simulink model "Buck_28V_12V_Analysis"  (R2023a)
settings: Solver=ode23t  StartTime=0.0  StopTime=0.05  MaxStep=1e-6  RelTol=1e-3
undefined symbols (not defined in the file): Rload
libraries: ee_lib x34, nesl_utility x33, fl_lib x26, simulink x24, slpidlib x4, simulink_extras x3
(part 2 of 2)

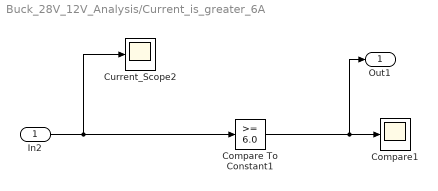
== system Buck_28V_12V_Analysis/Current_is_greater_6A ==
  In2 : Inport
  Compare To Constant1 : simulink/Logic and Bit Operations/Compare To Constant  relop=>=  const=6.0  OutDataTypeStr=boolean  ZeroCross=off
  Compare1 : Scope
  Current_Scope2 : Scope
  Out1 : Outport
  wires:
  Compare To Constant1/1 -> Out1/1, Compare1/1
  In2/1 -> Compare To Constant1/1, Current_Scope2/1

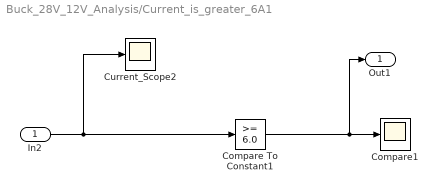
== system Buck_28V_12V_Analysis/Current_is_greater_6A1 ==
  In2 : Inport
  Compare To Constant1 : simulink/Logic and Bit Operations/Compare To Constant  relop=>=  const=6.0  OutDataTypeStr=boolean  ZeroCross=off
  Compare1 : Scope
  Current_Scope2 : Scope
  Out1 : Outport
  wires:
  In2/1 -> Current_Scope2/1, Compare To Constant1/1
  Compare To Constant1/1 -> Compare1/1, Out1/1

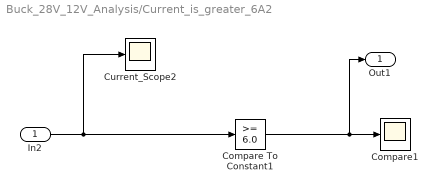
== system Buck_28V_12V_Analysis/Current_is_greater_6A2 ==
  In2 : Inport
  Compare To Constant1 : simulink/Logic and Bit Operations/Compare To Constant  relop=>=  const=6.0  OutDataTypeStr=boolean  ZeroCross=off
  Compare1 : Scope
  Current_Scope2 : Scope
  Out1 : Outport
  wires:
  In2/1 -> Current_Scope2/1, Compare To Constant1/1
  Compare To Constant1/1 -> Compare1/1, Out1/1

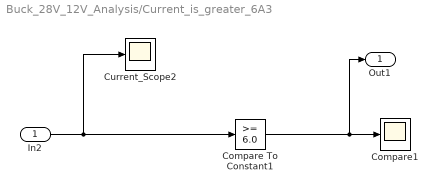
== system Buck_28V_12V_Analysis/Current_is_greater_6A3 ==
  In2 : Inport
  Compare To Constant1 : simulink/Logic and Bit Operations/Compare To Constant  relop=>=  const=6.0  OutDataTypeStr=boolean  ZeroCross=off
  Compare1 : Scope
  Current_Scope2 : Scope
  Out1 : Outport
  wires:
  In2/1 -> Current_Scope2/1, Compare To Constant1/1
  Compare To Constant1/1 -> Compare1/1, Out1/1

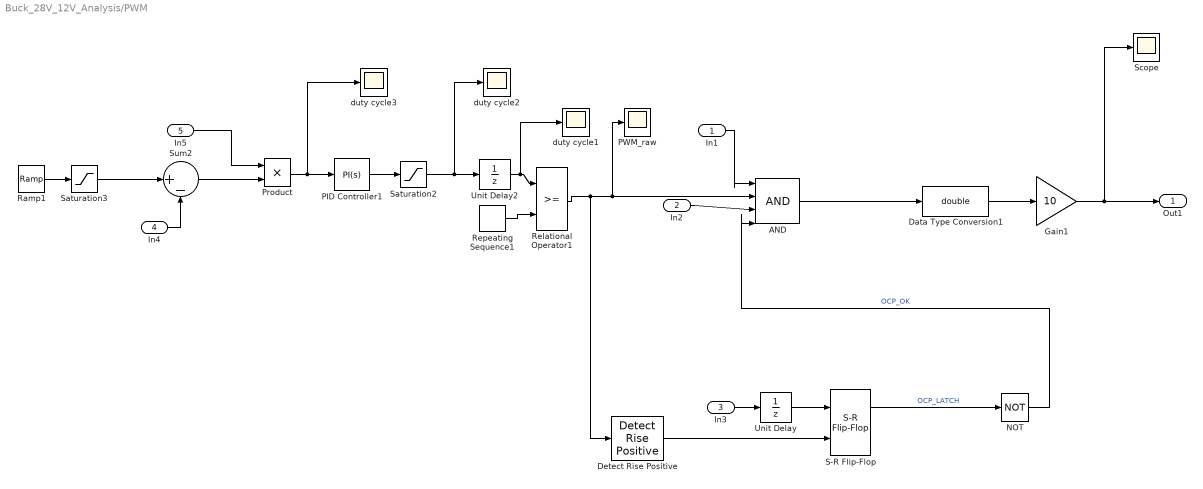
== system Buck_28V_12V_Analysis/PWM ==
  In1 : Inport
  In2 : Inport  Port=2
  In3 : Inport  Port=3
  In4 : Inport  Port=4
  In5 : Inport  Port=5
  AND : Logic  Inputs=4  IconShape=distinctive  AllPortsSameDT=off  OutDataTypeStr=boolean
  Data Type Conversion1 : DataTypeConversion  OutDataTypeStr=double  SaturateOnIntegerOverflow=off  RndMeth=Floor
  Detect Rise Positive : simulink/Logic and Bit Operations/Detect Rise Positive  vinit=0  OutDataTypeStr=boolean
  Gain1 : Gain  Gain=10
  NOT : Logic  Operator=NOT  IconShape=distinctive  AllPortsSameDT=off  OutDataTypeStr=boolean
  PID Controller1 : slpidlib/PID Controller  Controller=PI  Form=Parallel  TimeDomain=Continuous-time  UseExternalTs=off  SampleTime=-1  IntegratorMethod=Forward Euler  FilterMethod=Forward Euler  ControllerParametersSource=internal  P=0.02  I=50  UseKiTs=off  D=0  N=100  UseFilter=on  TunerSelectOption=Transfer Function Based (PID Tuner App)  ZeroCross=off  InitialConditionSource=internal  InitialConditionForIntegrator=0  InitialConditionForFilter=0  DifferentiatorICPrevScaledInput=0  ExternalReset=none  TrackingMode=off  Kt=1  LimitOutput=off  SatLimitsSource=internal  UpperSaturationLimit=inf  LowerSaturationLimit=-inf  LinearizeAsGain=on  AntiWindupMode=none  Kb=1  LimitIntegrator=off  UpperIntegratorSaturationLimit=inf  LowerIntegratorSaturationLimit=-inf  POutMin=[]  POutMax=[]  IOutMin=[]  IOutMax=[]  DOutMin=[]  DOutMax=[]  NOutMin=[]  NOutMax=[]  SumOutMin=[]  SumOutMax=[]  SaturationOutMin=[]  SaturationOutMax=[]  PParamMin=[]  PParamMax=[]  IParamMin=[]  IParamMax=[]  DParamMin=[]  DParamMax=[]  NParamMin=[]  NParamMax=[]  KbParamMin=[]  KbParamMax=[]  KtParamMin=[]  KtParamMax=[]  KbOutMin=[]  KbOutMax=[]  KtOutMin=[]  KtOutMax=[]  IntegratorOutMin=[]  IntegratorOutMax=[]  FilterOutMin=[]  FilterOutMax=[]  SumI1OutMin=[]  SumI1OutMax=[]  SumI2OutMin=[]  SumI2OutMax=[]  SumI3OutMin=[]  SumI3OutMax=[]  SumI4OutMin=[]  SumI4OutMax=[]  SumDOutMin=[]  SumDOutMax=[]  DifferentiatorOutMin=[]  DifferentiatorOutMax=[]  FilterDiffOutCoefMin=[]  FilterDiffOutCoefMax=[]  ReciprocalOutMin=[]  ReciprocalOutMax=[]  SumDenOutMin=[]  SumDenOutMax=[]  SumNumOutMin=[]  SumNumOutMax=[]  DivideOutMin=[]  DivideOutMax=[]  UdiffTsProdOutMin=[]  UdiffTsProdOutMax=[]  NTsProdOutMin=[]  NTsProdOutMax=[]  UintegralTsProdOutMin=[]  UintegralTsProdOutMax=[]  UngainTsProdOutMin=[]  UngainTsProdOutMax=[]  ClampingZeroOutDataTypeStr=Inherit: Inherit via back propagation  ClampingZeroOutMin=[]  ClampingZeroOutMax=[]  FilterDenConstantOutDataTypeStr=Inherit: Inherit via back propagation  FilterDenConstantOutMin=[]  FilterDenConstantOutMax=[]  PCopyOutDataTypeStr=Inherit: Inherit via back propagation  PCopyOutMin=[]  PCopyOutMax=[]  NCopyOutDataTypeStr=Inherit: Inherit via back propagation  NCopyOutMin=[]  NCopyOutMax=[]  IntegratorContinuousStateAttributes=''  IntegratorStateMustResolveToSignalObject=off  IntegratorRTWStateStorageClass=Auto  FilterContinuousStateAttributes=''  FilterStateMustResolveToSignalObject=off  FilterRTWStateStorageClass=Auto  ParallelPVariant=InternalParameters  IdealPVariant=Disabled  IVariant=InternalParameters  DVariant=Disabled  IntegratorVariant=Continuous  SatVariant=Disabled  AWVariant=Passthrough  PCopyVariant=Disabled  TRVariant=Disabled  FdbkBlocksVariant=Forward  IdealPFdbkVariant=Disabled  SatFdbkVariant=Disabled  DerivativeFilterVariant=Disabled  NVariant=Disabled  NCopyVariant=Disabled_SignalSpec  FilterICVariant=Disabled  IntegratorICVariant=InternalICs  ExternalResetVariant=Disabled  TRSumVariant=Passthrough  SumFdbkVariant=Disabled  SumVariant=Sum_PI  TsampFilterVariant=InternalTs  TsampNgainVariant=Passthrough  TsampIntegralVariant=Disabled_SignalSpec  ExternalSaturationOutDataTypeStr=Inherit: Same as second input
  PWM_raw : Scope
  Product : Product
  Ramp1 : simulink/Sources/Ramp  slope=6000  start=0  InitialOutput=0
  Relational Operator1 : RelationalOperator  OutDataTypeStr=boolean  RndMeth=Simplest  InputSameDT=off
  Repeating Sequence1 : simulink/Sources/Repeating Sequence  rep_seq_t=[0 10e-6]  rep_seq_y=[0 1]
  S-R Flip-Flop : simulink_extras/Flip Flops/S-R Flip-Flop  initial_condition=0
  Saturation2 : Saturate  UpperLimit=0.8  LowerLimit=0  ZeroCross=off
  Saturation3 : Saturate  UpperLimit=12  LowerLimit=0  ZeroCross=off
  Scope : Scope
  Sum2 : Sum  Inputs=|+-
  Unit Delay : UnitDelay  SampleTime=1e-7  HasFrameUpgradeWarning=on
  Unit Delay2 : UnitDelay  SampleTime=-1  HasFrameUpgradeWarning=on
  duty cycle1 : Scope
  duty cycle2 : Scope
  duty cycle3 : Scope
  Out1 : Outport
  wires:
  PID Controller1/1 -> Saturation2/1
  Unit Delay2/1 -> Relational Operator1/1, duty cycle1/1
  Saturation3/1 -> Sum2/1
  Ramp1/1 -> Saturation3/1
  Repeating Sequence1/1 -> Relational Operator1/2
  Sum2/1 -> Product/2
  Relational Operator1/1 -> AND/2, PWM_raw/1, Detect Rise Positive/1
  AND/1 -> Data Type Conversion1/1
  Data Type Conversion1/1 -> Gain1/1
  In1/1 -> AND/1
  In2/1 -> AND/3
  Gain1/1 -> Scope/1, Out1/1
  In4/1 -> Sum2/2
  In3/1 -> Unit Delay/1
  Detect Rise Positive/1 -> S-R Flip-Flop/2
  S-R Flip-Flop/1 -> NOT/1  "OCP_LATCH"
  NOT/1 -> AND/4  "OCP_OK"
  Unit Delay/1 -> S-R Flip-Flop/1
  Saturation2/1 -> duty cycle2/1, Unit Delay2/1
  In5/1 -> Product/1
  Product/1 -> duty cycle3/1, PID Controller1/1

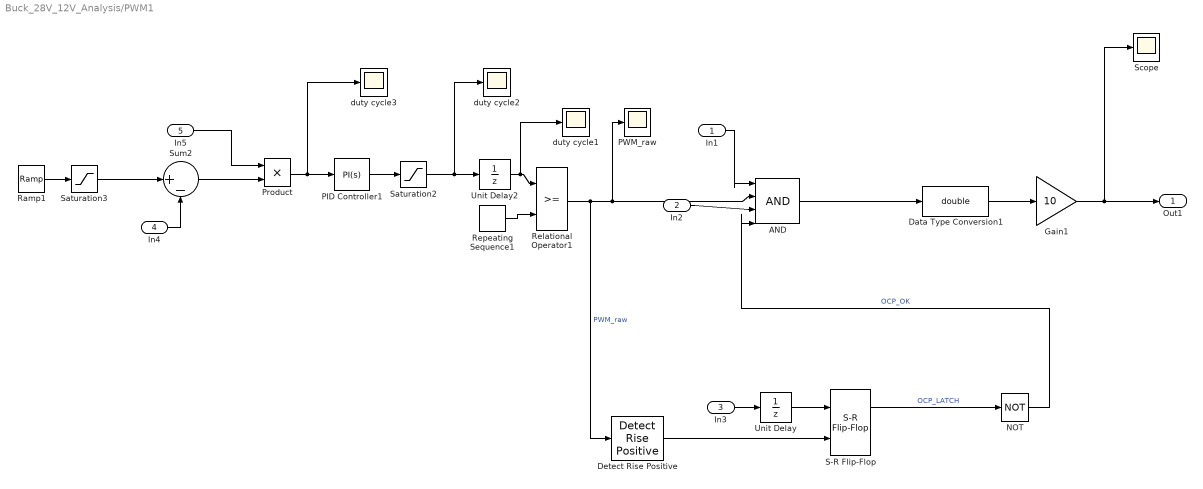
== system Buck_28V_12V_Analysis/PWM1 ==
  In1 : Inport
  In2 : Inport  Port=2
  In3 : Inport  Port=3
  In4 : Inport  Port=4
  In5 : Inport  Port=5
  AND : Logic  Inputs=4  IconShape=distinctive  AllPortsSameDT=off  OutDataTypeStr=boolean
  Data Type Conversion1 : DataTypeConversion  OutDataTypeStr=double  SaturateOnIntegerOverflow=off  RndMeth=Floor
  Detect Rise Positive : simulink/Logic and Bit Operations/Detect Rise Positive  vinit=0  OutDataTypeStr=boolean
  Gain1 : Gain  Gain=10
  NOT : Logic  Operator=NOT  IconShape=distinctive  AllPortsSameDT=off  OutDataTypeStr=boolean
  PID Controller1 : slpidlib/PID Controller  Controller=PI  Form=Parallel  TimeDomain=Continuous-time  UseExternalTs=off  SampleTime=-1  IntegratorMethod=Forward Euler  FilterMethod=Forward Euler  ControllerParametersSource=internal  P=0.003  I=55.8546  UseKiTs=off  D=0  N=100  UseFilter=on  TunerSelectOption=Transfer Function Based (PID Tuner App)  ZeroCross=off  InitialConditionSource=internal  InitialConditionForIntegrator=0  InitialConditionForFilter=0  DifferentiatorICPrevScaledInput=0  ExternalReset=none  TrackingMode=off  Kt=1  LimitOutput=off  SatLimitsSource=internal  UpperSaturationLimit=inf  LowerSaturationLimit=-inf  LinearizeAsGain=on  AntiWindupMode=none  Kb=1  LimitIntegrator=off  UpperIntegratorSaturationLimit=inf  LowerIntegratorSaturationLimit=-inf  POutMin=[]  POutMax=[]  IOutMin=[]  IOutMax=[]  DOutMin=[]  DOutMax=[]  NOutMin=[]  NOutMax=[]  SumOutMin=[]  SumOutMax=[]  SaturationOutMin=[]  SaturationOutMax=[]  PParamMin=[]  PParamMax=[]  IParamMin=[]  IParamMax=[]  DParamMin=[]  DParamMax=[]  NParamMin=[]  NParamMax=[]  KbParamMin=[]  KbParamMax=[]  KtParamMin=[]  KtParamMax=[]  KbOutMin=[]  KbOutMax=[]  KtOutMin=[]  KtOutMax=[]  IntegratorOutMin=[]  IntegratorOutMax=[]  FilterOutMin=[]  FilterOutMax=[]  SumI1OutMin=[]  SumI1OutMax=[]  SumI2OutMin=[]  SumI2OutMax=[]  SumI3OutMin=[]  SumI3OutMax=[]  SumI4OutMin=[]  SumI4OutMax=[]  SumDOutMin=[]  SumDOutMax=[]  DifferentiatorOutMin=[]  DifferentiatorOutMax=[]  FilterDiffOutCoefMin=[]  FilterDiffOutCoefMax=[]  ReciprocalOutMin=[]  ReciprocalOutMax=[]  SumDenOutMin=[]  SumDenOutMax=[]  SumNumOutMin=[]  SumNumOutMax=[]  DivideOutMin=[]  DivideOutMax=[]  UdiffTsProdOutMin=[]  UdiffTsProdOutMax=[]  NTsProdOutMin=[]  NTsProdOutMax=[]  UintegralTsProdOutMin=[]  UintegralTsProdOutMax=[]  UngainTsProdOutMin=[]  UngainTsProdOutMax=[]  ClampingZeroOutDataTypeStr=Inherit: Inherit via back propagation  ClampingZeroOutMin=[]  ClampingZeroOutMax=[]  FilterDenConstantOutDataTypeStr=Inherit: Inherit via back propagation  FilterDenConstantOutMin=[]  FilterDenConstantOutMax=[]  PCopyOutDataTypeStr=Inherit: Inherit via back propagation  PCopyOutMin=[]  PCopyOutMax=[]  NCopyOutDataTypeStr=Inherit: Inherit via back propagation  NCopyOutMin=[]  NCopyOutMax=[]  IntegratorContinuousStateAttributes=''  IntegratorStateMustResolveToSignalObject=off  IntegratorRTWStateStorageClass=Auto  FilterContinuousStateAttributes=''  FilterStateMustResolveToSignalObject=off  FilterRTWStateStorageClass=Auto  ParallelPVariant=InternalParameters  IdealPVariant=Disabled  IVariant=InternalParameters  DVariant=Disabled  IntegratorVariant=Continuous  SatVariant=Disabled  AWVariant=Passthrough  PCopyVariant=Disabled  TRVariant=Disabled  FdbkBlocksVariant=Forward  IdealPFdbkVariant=Disabled  SatFdbkVariant=Disabled  DerivativeFilterVariant=Disabled  NVariant=Disabled  NCopyVariant=Disabled_SignalSpec  FilterICVariant=Disabled  IntegratorICVariant=InternalICs  ExternalResetVariant=Disabled  TRSumVariant=Passthrough  SumFdbkVariant=Disabled  SumVariant=Sum_PI  TsampFilterVariant=InternalTs  TsampNgainVariant=Passthrough  TsampIntegralVariant=Disabled_SignalSpec  ExternalSaturationOutDataTypeStr=Inherit: Same as second input
  PWM_raw : Scope
  Product : Product
  Ramp1 : simulink/Sources/Ramp  slope=6000  start=0  InitialOutput=0
  Relational Operator1 : RelationalOperator  OutDataTypeStr=boolean  RndMeth=Simplest  InputSameDT=off
  Repeating Sequence1 : simulink/Sources/Repeating Sequence  rep_seq_t=[0 10e-6]  rep_seq_y=[0 1]
  S-R Flip-Flop : simulink_extras/Flip Flops/S-R Flip-Flop  initial_condition=0
  Saturation2 : Saturate  UpperLimit=0.8  LowerLimit=0  ZeroCross=off
  Saturation3 : Saturate  UpperLimit=12  LowerLimit=0  ZeroCross=off
  Scope : Scope
  Sum2 : Sum  Inputs=|+-
  Unit Delay : UnitDelay  SampleTime=1e-7  HasFrameUpgradeWarning=on
  Unit Delay2 : UnitDelay  SampleTime=-1  HasFrameUpgradeWarning=on
  duty cycle1 : Scope
  duty cycle2 : Scope
  duty cycle3 : Scope
  Out1 : Outport
  wires:
  PID Controller1/1 -> Saturation2/1
  Unit Delay2/1 -> Relational Operator1/1, duty cycle1/1
  Saturation3/1 -> Sum2/1
  Ramp1/1 -> Saturation3/1
  Repeating Sequence1/1 -> Relational Operator1/2
  Sum2/1 -> Product/2
  Relational Operator1/1 -> PWM_raw/1, AND/2, Detect Rise Positive/1  "PWM_raw"
  AND/1 -> Data Type Conversion1/1
  Data Type Conversion1/1 -> Gain1/1
  In1/1 -> AND/1
  In2/1 -> AND/3
  Gain1/1 -> Scope/1, Out1/1
  In4/1 -> Sum2/2
  In3/1 -> Unit Delay/1
  Detect Rise Positive/1 -> S-R Flip-Flop/2
  S-R Flip-Flop/1 -> NOT/1  "OCP_LATCH"
  NOT/1 -> AND/4  "OCP_OK"
  Unit Delay/1 -> S-R Flip-Flop/1
  Saturation2/1 -> duty cycle2/1, Unit Delay2/1
  In5/1 -> Product/1
  Product/1 -> duty cycle3/1, PID Controller1/1

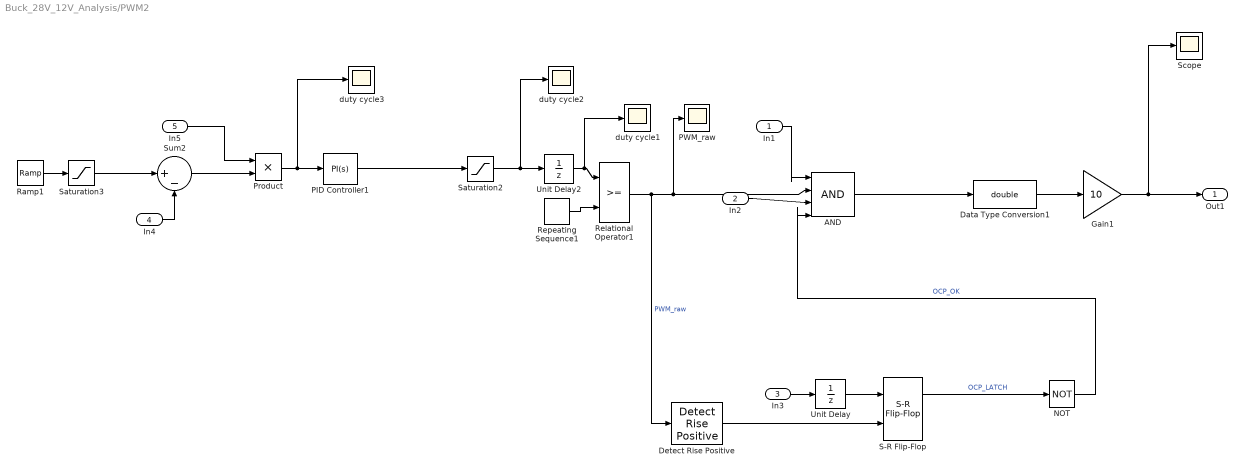
== system Buck_28V_12V_Analysis/PWM2 ==
  In1 : Inport
  In2 : Inport  Port=2
  In3 : Inport  Port=3
  In4 : Inport  Port=4
  In5 : Inport  Port=5
  AND : Logic  Inputs=4  IconShape=distinctive  AllPortsSameDT=off  OutDataTypeStr=boolean
  Data Type Conversion1 : DataTypeConversion  OutDataTypeStr=double  SaturateOnIntegerOverflow=off  RndMeth=Floor
  Detect Rise Positive : simulink/Logic and Bit Operations/Detect Rise Positive  vinit=0  OutDataTypeStr=boolean
  Gain1 : Gain  Gain=10
  NOT : Logic  Operator=NOT  IconShape=distinctive  AllPortsSameDT=off  OutDataTypeStr=boolean
  PID Controller1 : slpidlib/PID Controller  Controller=PI  Form=Parallel  TimeDomain=Continuous-time  UseExternalTs=off  SampleTime=-1  IntegratorMethod=Forward Euler  FilterMethod=Forward Euler  ControllerParametersSource=internal  P=0.003  I=55.8546  UseKiTs=off  D=0  N=100  UseFilter=on  TunerSelectOption=Transfer Function Based (PID Tuner App)  ZeroCross=off  InitialConditionSource=internal  InitialConditionForIntegrator=0  InitialConditionForFilter=0  DifferentiatorICPrevScaledInput=0  ExternalReset=none  TrackingMode=off  Kt=1  LimitOutput=off  SatLimitsSource=internal  UpperSaturationLimit=inf  LowerSaturationLimit=-inf  LinearizeAsGain=on  AntiWindupMode=none  Kb=1  LimitIntegrator=off  UpperIntegratorSaturationLimit=inf  LowerIntegratorSaturationLimit=-inf  POutMin=[]  POutMax=[]  IOutMin=[]  IOutMax=[]  DOutMin=[]  DOutMax=[]  NOutMin=[]  NOutMax=[]  SumOutMin=[]  SumOutMax=[]  SaturationOutMin=[]  SaturationOutMax=[]  PParamMin=[]  PParamMax=[]  IParamMin=[]  IParamMax=[]  DParamMin=[]  DParamMax=[]  NParamMin=[]  NParamMax=[]  KbParamMin=[]  KbParamMax=[]  KtParamMin=[]  KtParamMax=[]  KbOutMin=[]  KbOutMax=[]  KtOutMin=[]  KtOutMax=[]  IntegratorOutMin=[]  IntegratorOutMax=[]  FilterOutMin=[]  FilterOutMax=[]  SumI1OutMin=[]  SumI1OutMax=[]  SumI2OutMin=[]  SumI2OutMax=[]  SumI3OutMin=[]  SumI3OutMax=[]  SumI4OutMin=[]  SumI4OutMax=[]  SumDOutMin=[]  SumDOutMax=[]  DifferentiatorOutMin=[]  DifferentiatorOutMax=[]  FilterDiffOutCoefMin=[]  FilterDiffOutCoefMax=[]  ReciprocalOutMin=[]  ReciprocalOutMax=[]  SumDenOutMin=[]  SumDenOutMax=[]  SumNumOutMin=[]  SumNumOutMax=[]  DivideOutMin=[]  DivideOutMax=[]  UdiffTsProdOutMin=[]  UdiffTsProdOutMax=[]  NTsProdOutMin=[]  NTsProdOutMax=[]  UintegralTsProdOutMin=[]  UintegralTsProdOutMax=[]  UngainTsProdOutMin=[]  UngainTsProdOutMax=[]  ClampingZeroOutDataTypeStr=Inherit: Inherit via back propagation  ClampingZeroOutMin=[]  ClampingZeroOutMax=[]  FilterDenConstantOutDataTypeStr=Inherit: Inherit via back propagation  FilterDenConstantOutMin=[]  FilterDenConstantOutMax=[]  PCopyOutDataTypeStr=Inherit: Inherit via back propagation  PCopyOutMin=[]  PCopyOutMax=[]  NCopyOutDataTypeStr=Inherit: Inherit via back propagation  NCopyOutMin=[]  NCopyOutMax=[]  IntegratorContinuousStateAttributes=''  IntegratorStateMustResolveToSignalObject=off  IntegratorRTWStateStorageClass=Auto  FilterContinuousStateAttributes=''  FilterStateMustResolveToSignalObject=off  FilterRTWStateStorageClass=Auto  ParallelPVariant=InternalParameters  IdealPVariant=Disabled  IVariant=InternalParameters  DVariant=Disabled  IntegratorVariant=Continuous  SatVariant=Disabled  AWVariant=Passthrough  PCopyVariant=Disabled  TRVariant=Disabled  FdbkBlocksVariant=Forward  IdealPFdbkVariant=Disabled  SatFdbkVariant=Disabled  DerivativeFilterVariant=Disabled  NVariant=Disabled  NCopyVariant=Disabled_SignalSpec  FilterICVariant=Disabled  IntegratorICVariant=InternalICs  ExternalResetVariant=Disabled  TRSumVariant=Passthrough  SumFdbkVariant=Disabled  SumVariant=Sum_PI  TsampFilterVariant=InternalTs  TsampNgainVariant=Passthrough  TsampIntegralVariant=Disabled_SignalSpec  ExternalSaturationOutDataTypeStr=Inherit: Same as second input
  PWM_raw : Scope
  Product : Product
  Ramp1 : simulink/Sources/Ramp  slope=6000  start=0  InitialOutput=0
  Relational Operator1 : RelationalOperator  OutDataTypeStr=boolean  RndMeth=Simplest  InputSameDT=off
  Repeating Sequence1 : simulink/Sources/Repeating Sequence  rep_seq_t=[0 10e-6]  rep_seq_y=[0 1]
  S-R Flip-Flop : simulink_extras/Flip Flops/S-R Flip-Flop  initial_condition=0
  Saturation2 : Saturate  UpperLimit=0.8  LowerLimit=0  ZeroCross=off
  Saturation3 : Saturate  UpperLimit=12  LowerLimit=0  ZeroCross=off
  Scope : Scope
  Sum2 : Sum  Inputs=|+-
  Unit Delay : UnitDelay  SampleTime=1e-7  HasFrameUpgradeWarning=on
  Unit Delay2 : UnitDelay  SampleTime=-1  HasFrameUpgradeWarning=on
  duty cycle1 : Scope
  duty cycle2 : Scope
  duty cycle3 : Scope
  Out1 : Outport
  wires:
  Unit Delay2/1 -> Relational Operator1/1, duty cycle1/1
  Saturation3/1 -> Sum2/1
  Ramp1/1 -> Saturation3/1
  Repeating Sequence1/1 -> Relational Operator1/2
  Sum2/1 -> Product/2
  Relational Operator1/1 -> PWM_raw/1, AND/2, Detect Rise Positive/1  "PWM_raw"
  AND/1 -> Data Type Conversion1/1
  Data Type Conversion1/1 -> Gain1/1
  In1/1 -> AND/1
  In2/1 -> AND/3
  Gain1/1 -> Scope/1, Out1/1
  In4/1 -> Sum2/2
  In3/1 -> Unit Delay/1
  Detect Rise Positive/1 -> S-R Flip-Flop/2
  S-R Flip-Flop/1 -> NOT/1  "OCP_LATCH"
  NOT/1 -> AND/4  "OCP_OK"
  Unit Delay/1 -> S-R Flip-Flop/1
  Saturation2/1 -> duty cycle2/1, Unit Delay2/1
  In5/1 -> Product/1
  Product/1 -> duty cycle3/1, PID Controller1/1
  PID Controller1/1 -> Saturation2/1
